simulink model "AWU_clamping"  (R2023a)
settings: Solver=VariableStepAuto  StartTime=0.0  StopTime=60  RelTol=1e-3
values from neighbouring files (symbols this model uses):
  lower_limit = -0.2    [AWU_system_data.sldd]
  upper_limit = 0.2    [AWU_system_data.sldd]
undefined symbols (not defined in the file or in its folder): DiscIntNeverNeededParam
libraries: simulink x1, SignalEditorBlockLib x1
settings Model: DataDictionary=AWU_system_data.sldd  Creator=tshintai  LastModifiedBy=tshintai
settings SolverCC: AlgebraicLoopSolver=TrustRegion
settings OptimizationCC: ReuseModelBlockBuffer=off
settings DebuggingCC: UnconnectedInputMsg=warning  UnconnectedOutputMsg=warning  UnconnectedLineMsg=warning
settings ModelReferenceCC: EnableRefExpFcnMdlSchedulingChecks=on
settings RTWCC: DLArmComputeVersion=19.05

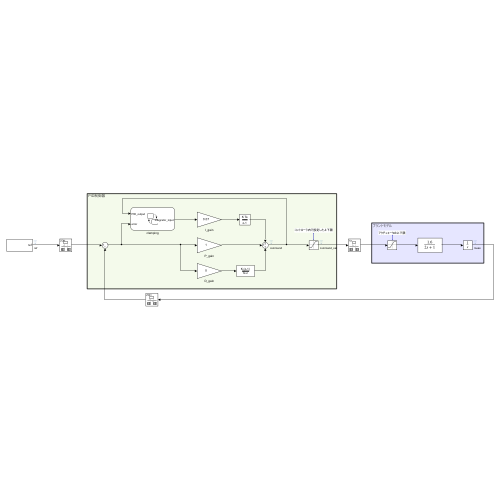
[thumbnail: Simulink's stored preview of the top-level diagram]
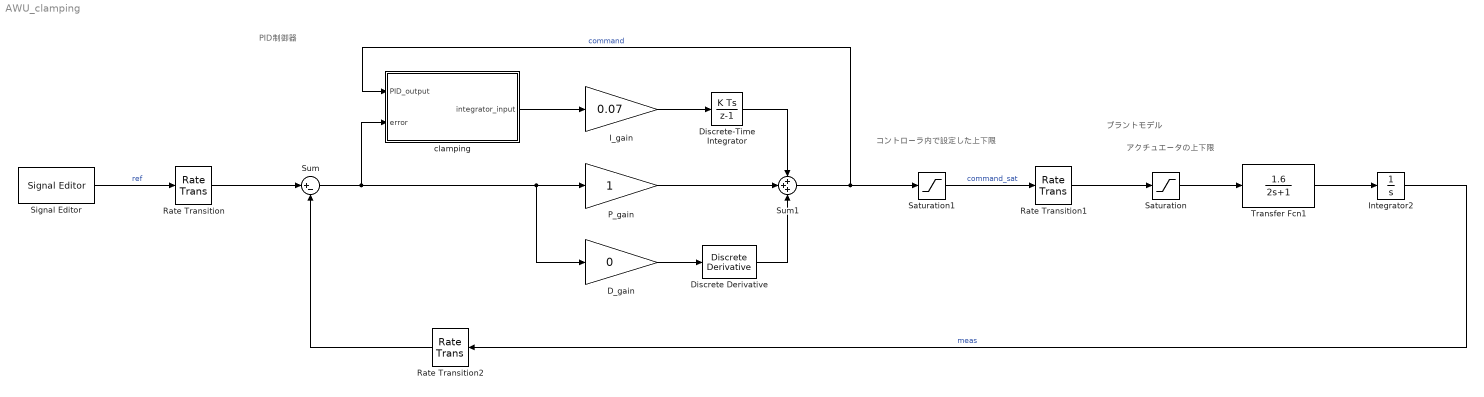
== system AWU_clamping ==
  note: PID制御器
  note: アクチュエータの上下限
  note: プラントモデル
  note: コントローラ内で設定した上下限
  D_gain : Gain  Gain=0
  Discrete Derivative : simulink/Discrete/Discrete Derivative  gainval=1.0  ICPrevScaledInput=0.0  OutMin=[]  OutMax=[]  OutDataType=fixdt(1, 16)  OutScaling=2^-10  DoSatur=off
  Discrete-Time Integrator : DiscreteIntegrator  SampleTime=-1  ICPrevOutput=DiscIntNeverNeededParam  ICPrevScaledInput=DiscIntNeverNeededParam
  I_gain : Gain  Gain=0.07
  Integrator2 : Integrator
  P_gain : Gain
  Rate Transition : RateTransition  OutPortSampleTime=TimeStep
  Rate Transition1 : RateTransition
  Rate Transition2 : RateTransition  OutPortSampleTime=TimeStep
  Saturation : Saturate  UpperLimit=0.2  LowerLimit=-0.2
  Saturation1 : Saturate  UpperLimit=upper_limit  LowerLimit=lower_limit
  Signal Editor : SignalEditorBlockLib/Signal Editor  FileName=AWU_ref_signal.mat  ActiveScenario=Scenario  ActiveSignal=ref  IsBus=off  OutputBusObjectStr=Bus: BusObject  SampleTime=0  ZeroCross=off  OutputAfterFinalValue=Holding final value  Unit=inherit  PreserveSignalName=on  ApplySigPropsToAllScenarios=on
  Sum : Sum  Inputs=|+-
  Sum1 : Sum  Inputs=+++
  Transfer Fcn1 : TransferFcn  Numerator=[1.6]  Denominator=[2 1]
  clamping : Stateflow chart  TreatAsAtomicUnit=on
  wires:
  Transfer Fcn1/1 -> Integrator2/1
  Saturation/1 -> Transfer Fcn1/1
  Integrator2/1 -> Rate Transition2/1  "meas"
  Sum/1 -> D_gain/1, P_gain/1, clamping/2(error)
  Discrete-Time Integrator/1 -> Sum1/1
  Sum1/1 -> clamping/1(PID_output), Saturation1/1  "command"
  D_gain/1 -> Discrete Derivative/1
  P_gain/1 -> Sum1/2
  Discrete Derivative/1 -> Sum1/3
  I_gain/1 -> Discrete-Time Integrator/1
  Saturation1/1 -> Rate Transition1/1  "command_sat"
  Signal Editor/1 -> Rate Transition/1  "ref"
  clamping/1(integrator_input) -> I_gain/1
  Rate Transition/1 -> Sum/1
  Rate Transition1/1 -> Saturation/1
  Rate Transition2/1 -> Sum/2

== stateflow chart AWU_clamping/clamping ==
  (default) -> (junction 4)
  (junction 4) -> (junction 9) [order 1] : [
      | PID_output > upper_limit
      | ]
  (junction 4) -> (junction 41) [order 2]
  (junction 9) -> (junction 11)
  (junction 41) -> (junction 13) [order 1] : [
      | PID_output < lower_limit
      | ]
  (junction 41) -> (junction 6) [order 2] : {
      | integrator_input = error;
      | }
  (junction 13) -> (junction 22)
  (junction 22) -> (junction 24) [order 1] : [
      | error < 0
      | ]
  (junction 11) -> (junction 17) [order 1] : [
      | error > 0
      | ]
  (junction 22) -> (junction 33) [order 2] : {
      | integrator_input = error;
      | }
  (junction 24) -> (junction 36) : {
      | integrator_input = 0;
      | }
  (junction 11) -> (junction 29) [order 2] : {
      | integrator_input = error;
      | }
  (junction 17) -> (junction 19) : {
      | integrator_input = 0;
      | }
  (junction 33) -> (junction 6)
  (junction 36) -> (junction 33)
  (junction 29) -> (junction 36)
  (junction 19) -> (junction 29)
  (junction 6) -> (junction 39)
  data: PID_output input; error input; integrator_input output; lower_limit parameter; upper_limit parameter
